simulink model "appendix01_Bicopter_OpenLoop"  (R2026b)
settings: Solver=FixedStepAuto  StopTime=inf  EnableMultiTasking=on
undefined symbols (not defined in the file or in its folder): dspblkCoreblockFVToolHelper, gcbh, ODR
libraries: arduinolib x6, arduinowifilib x2, arduinosensorlib x1
settings Model: SILPILModeSetting=veronly  Creator=lcree  LastModifiedBy=ayeo
settings OptimizationCC: DifferentSizesBufferReuse=on  EnhancedBackFolding=on  MaxStackSize=64  OptimizationCustomize=off  OptimizeBlockOrder=speed
settings DebuggingCC: ParameterTunabilityLossMsg=error
settings HardwareCC: ProdHWDeviceType=ARM Compatible->ARM Cortex  ProdLargestAtomicFloat=Double  ProdLargestAtomicInteger=Long  UseEmbeddedCoderFeatures=off  UseSimulinkCoderFeatures=off
settings SFSimCC: MATLABDynamicMemAlloc=off
settings RTWCC: BuildConfiguration=Faster Runs  Description=Embedded Coder  HardwareBoard=Arduino Nano 33 IoT  SystemTargetFile=ert.tlc  TLCOptions=-aInlineSetEventsForThisBaseRateFcn=TLC_FALSE -aSuppressMultiTaskScheduler=TLC_FALSE -aRateBasedStepFcn=1  TemplateMakefile=ert_default_tmf  Toolchain=Arduino ARM
settings CodeAppCC: ForceParamTrailComments=on  OperatorAnnotations=on
settings ERTTargetCC: DynamicArrayContainerType=coder::array  ERTCustomFileBanners=off  ExtModeIntrfLevel=Level2 - Open  ExtModeMexFile=ext_xcp  ExtModeStaticAlloc=on  ModelStepFunctionPrototypeControlCompliant=off  SupportContinuousTime=on  SupportNonInlinedSFcns=on  SupportVariableSizeSignals=on

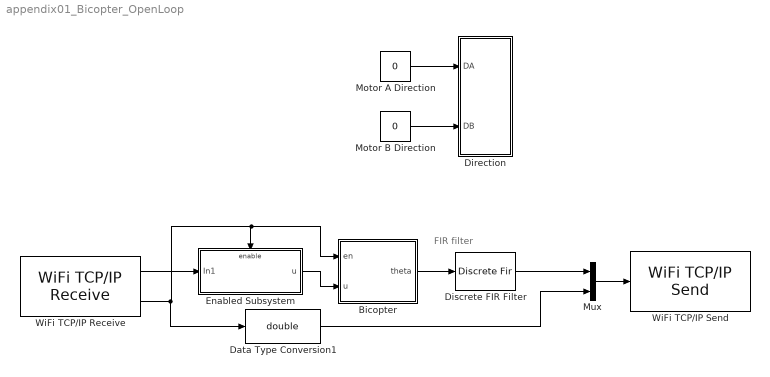
== system appendix01_Bicopter_OpenLoop ==
  note: FIR filter
  Bicopter : Subsystem
  Data Type Conversion1 : DataTypeConversion  OutDataTypeStr=double  SaturateOnIntegerOverflow=off  RndMeth=Floor
  Direction : Subsystem
  Discrete FIR Filter : DiscreteFir  LoadFcn=dspblkCoreblockFVToolHelper(gcbh,'load');  Coefficients=0.1*ones(1,10)  OutDataTypeStr=Inherit: Same as accumulator
      settings: CopyFcn=dspblkCoreblockFVToolHelper(gcbh,'copy');  DeleteFcn=dspblkCoreblockFVToolHelper(gcbh,'close');  ModelCloseFcn=dspblkCoreblockFVToolHelper(gcbh,'close');  PreSaveFcn=dspblkCoreblockFVToolHelper(gcbh,'presave');  PostSaveFcn=dspblkCoreblockFVToolHelper(gcbh,'postsave');  CloseFcn=dspblkCoreblockFVToolHelper(gcbh,'close');
  Enabled Subsystem : Subsystem  TreatAsAtomicUnit=on
  Motor A Direction : Constant  Value=0  OutDataTypeStr=boolean
  Motor B Direction : Constant  Value=0  OutDataTypeStr=boolean
  Mux : Mux  Inputs=2
  WiFi TCP/IP Receive : arduinowifilib/WiFi TCP//IP Receive  Mode_=Server  serverport=25000  RemoteAddr_=192.168.1.2  RemoteServerPort_=25000  DataType_=int8  DataSize_=1  SampleTime_=0.01  remoteipoctet1=192  remoteipoctet2=168  remoteipoctet3=1  remoteipoctet4=2  wifiTCPServerIndex=0  wifiTCPClientIndex=0  blockPlatform=ARDUINO  isARMArch=true  BlockingMode_=off  BlockTimeout_=1
  WiFi TCP/IP Send : arduinowifilib/WiFi TCP//IP Send  Mode_=Server  serverport=25000  RemoteAddr_=192.168.1.2  RemoteServerPort_=25000  remoteipoctet1=192  remoteipoctet2=168  remoteipoctet3=1  remoteipoctet4=2  wifiTCPServerIndex=0  wifiTCPClientIndex=0  blockPlatform=ARDUINO  isARMArch=true
  wires:
  Motor A Direction/1 -> Direction/1(DA)
  Motor B Direction/1 -> Direction/2(DB)
  WiFi TCP/IP Receive/1 -> Enabled Subsystem/1(In1)
  WiFi TCP/IP Receive/2 -> Data Type Conversion1/1, Bicopter/1(en), Enabled Subsystem/Enable
  Mux/1 -> WiFi TCP/IP Send/1
  Data Type Conversion1/1 -> Mux/2
  Enabled Subsystem/1(u) -> Bicopter/2(u)
  Bicopter/1(theta) -> Discrete FIR Filter/1
  Discrete FIR Filter/1 -> Mux/1

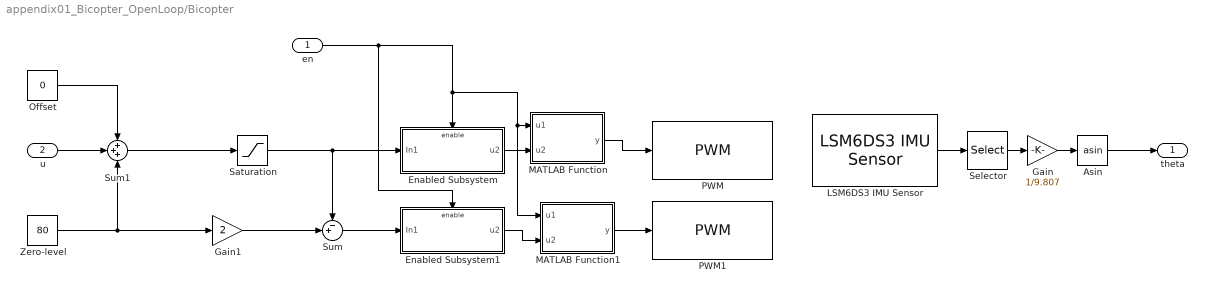
== system appendix01_Bicopter_OpenLoop/Bicopter ==
  en : Inport
  u : Inport  Port=2
  Asin : Trigonometry  Operator=asin
  Enabled Subsystem : Subsystem  TreatAsAtomicUnit=on
  Enabled Subsystem1 : Subsystem  TreatAsAtomicUnit=on
  Gain : Gain  Gain=1/9.807
  Gain1 : Gain  Gain=2
  LSM6DS3 IMU Sensor : arduinosensorlib/LSM6DS3 IMU Sensor  I2CModule=0  I2CAddress=0x6A  IsActiveAcceleration=on  IsActiveAngularRate=off  IsActiveTemperature=off  IsActiveStatus=off  IsActiveTimeStamp=off  spf=1  SampleTime=0.01  QueueSizeFactor=1  AccelerometerRange=+/- 2g  AccelerometerODR=208 Hz  SelectAnalogBW=off  AccelLPF1BW=400 Hz  AccelSelectCompositeFilter=Low pass filter  AccelLPF2BW=ODR/400  AccelHPFBW=ODR/100  GyroscopeRange=250 dps  GyroscopeODR=12.5 Hz  SelectGyroscopeHPF=off  GyroHPFBW=0.0081 Hz
  MATLAB Function : MATLAB Function  TreatAsAtomicUnit=on
  MATLAB Function1 : MATLAB Function  TreatAsAtomicUnit=on
  Offset : Constant  Value=0
  PWM : arduinolib/PWM  pinNumber=5  frequencyType=Default  desiredFrequency=490.2  achievableFrequency=490.2
  PWM1 : arduinolib/PWM  pinNumber=6  frequencyType=Default  desiredFrequency=490.2  achievableFrequency=490.2
  Saturation : Saturate  UpperLimit=255  LowerLimit=0  OutDataTypeStr=uint8
  Selector : Selector  InputPortWidth=3  IndexOptions=Index vector (dialog)  Indices=[1]  OutputSizes=1  RuntimeRangeChecks=off
  Sum : Sum  Inputs=-+|  OutDataTypeStr=uint8
  Sum1 : Sum  Inputs=+++
  Zero-level : Constant  Value=80
  theta : Outport
  wires:
  LSM6DS3 IMU Sensor/1 -> Selector/1
  Selector/1 -> Gain/1
  Gain1/1 -> Sum/2
  Gain/1 -> Asin/1
  Asin/1 -> theta/1
  Zero-level/1 -> Sum1/3, Gain1/1
  u/1 -> Sum1/2
  Offset/1 -> Sum1/1
  Sum1/1 -> Saturation/1
  Saturation/1 -> Enabled Subsystem/1(In1), Sum/1
  Sum/1 -> Enabled Subsystem1/1(In1)
  en/1 -> MATLAB Function1/1(u1), MATLAB Function/1(u1), Enabled Subsystem/Enable, Enabled Subsystem1/Enable
  Enabled Subsystem/1(u2) -> MATLAB Function/2(u2)
  MATLAB Function/1(y) -> PWM/1
  MATLAB Function1/1(y) -> PWM1/1
  Enabled Subsystem1/1(u2) -> MATLAB Function1/2(u2)

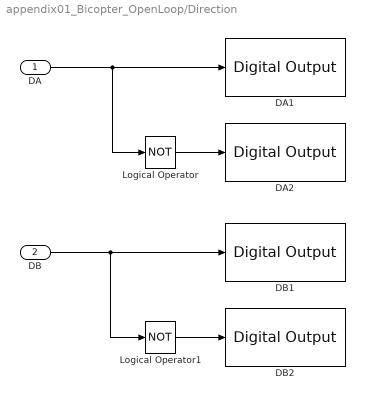
== system appendix01_Bicopter_OpenLoop/Direction ==
  DA : Inport
  DB : Inport  Port=2
  DA1 : arduinolib/Digital Output  pinNumber=8  Direction=output  blockPlatform=arduino
  DA2 : arduinolib/Digital Output  pinNumber=7  Direction=output  blockPlatform=arduino
  DB1 : arduinolib/Digital Output  pinNumber=3  Direction=output  blockPlatform=arduino
  DB2 : arduinolib/Digital Output  pinNumber=2  Direction=output  blockPlatform=arduino
  Logical Operator : Logic  Operator=NOT  IconShape=distinctive  AllPortsSameDT=off  OutDataTypeStr=boolean
  Logical Operator1 : Logic  Operator=NOT  IconShape=distinctive  AllPortsSameDT=off  OutDataTypeStr=boolean
  wires:
  DB/1 -> Logical Operator1/1, DB1/1
  DA/1 -> Logical Operator/1, DA1/1
  Logical Operator/1 -> DA2/1
  Logical Operator1/1 -> DB2/1

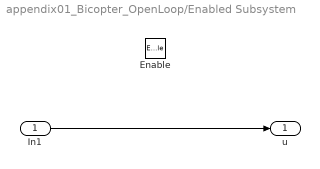
== system appendix01_Bicopter_OpenLoop/Enabled Subsystem ==
  In1 : Inport
  Enable : EnablePort
  u : Outport
  wires:
  In1/1 -> u/1

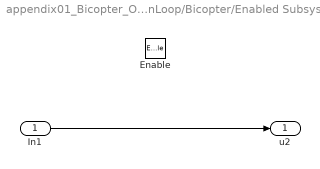
== system appendix01_Bicopter_OpenLoop/Bicopter/Enabled Subsystem ==
  In1 : Inport
  Enable : EnablePort  StatesWhenEnabling=reset
  u2 : Outport
  wires:
  In1/1 -> u2/1

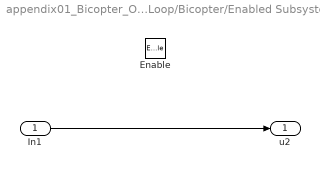
== system appendix01_Bicopter_OpenLoop/Bicopter/Enabled Subsystem1 ==
  In1 : Inport
  Enable : EnablePort  StatesWhenEnabling=reset
  u2 : Outport
  wires:
  In1/1 -> u2/1

== matlab function appendix01_Bicopter_OpenLoop/Bicopter/MATLAB Function1 ==
  data: u1 input; y output; u2 input
function y  = fcn(u1,u2)
y=uint8(0);
if u1 == 1
    y=uint8(u2);
end

== matlab function appendix01_Bicopter_OpenLoop/Bicopter/MATLAB Function ==
  data: u1 input; y output; u2 input
function y  = fcn(u1,u2)
y=uint8(0);
if u1 == 1
    y=uint8(u2);
end
